simulink model "second_graph_oct9"  (R2026a)
settings: Solver=VariableStepAuto
libraries: fl_lib x10, nesl_utility x7
settings Model: Creator=cathynguyen  LastModifiedBy=cathynguyen

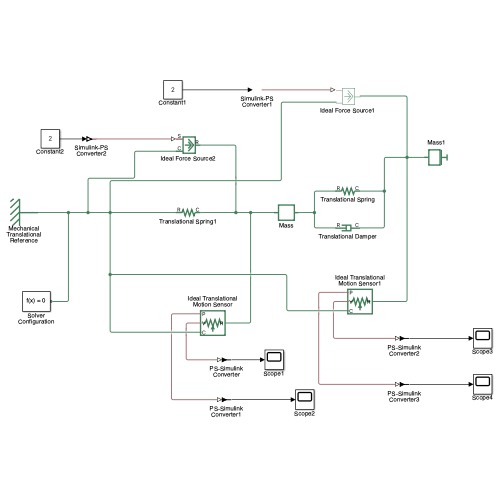
[thumbnail: Simulink's stored preview of the top-level diagram]
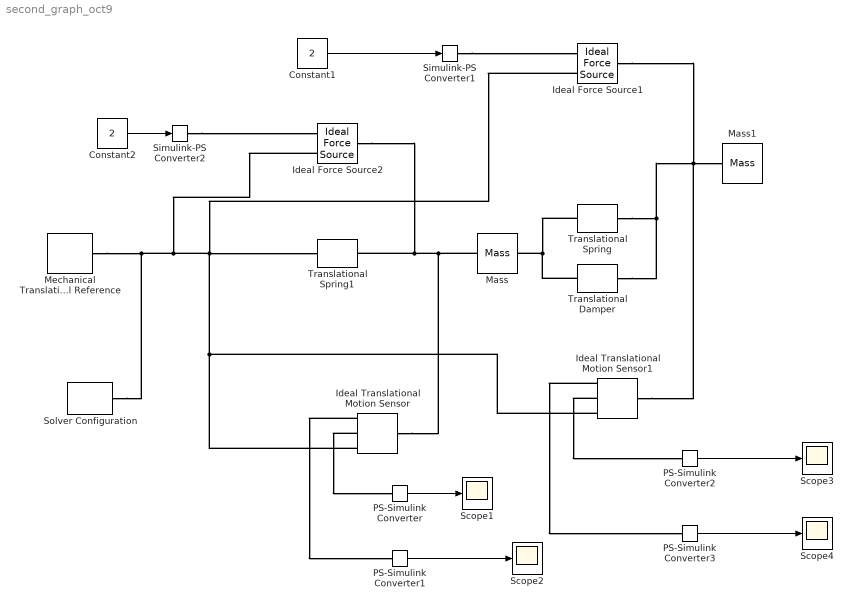
== system second_graph_oct9 ==
  Constant1 : Constant  Value=2
  Constant2 : Constant  Value=2
  Ideal Force Source1 : fl_lib/Mechanical/Mechanical Sources/Ideal Force Source
  Ideal Force Source2 : fl_lib/Mechanical/Mechanical Sources/Ideal Force Source
  Ideal Translational Motion Sensor : fl_lib/Mechanical/Mechanical Sensors/Ideal Translational Motion Sensor  reference=foundation.enum.MeasurementReference.difference  acceleration_port=false  velocity_port=true  position_port=true  offset=0 m
  Ideal Translational Motion Sensor1 : fl_lib/Mechanical/Mechanical Sensors/Ideal Translational Motion Sensor  reference=foundation.enum.MeasurementReference.difference  acceleration_port=false  velocity_port=true  position_port=true  offset=0 m
  Mass : fl_lib/Mechanical/Translational Elements/Mass  mass=1 kg  num_ports=foundation.enum.numPorts2.two  v_specify=off  v_priority=High  v=0 m/s  v_nominal_specify=off  v_nominal_value=1  v_nominal_unit=m/s  f_specify=off  f_priority=None  f=0 N  f_nominal_specify=off  f_nominal_value=1  f_nominal_unit=N
  Mass1 : fl_lib/Mechanical/Translational Elements/Mass  mass=1 kg  num_ports=foundation.enum.numPorts2.one  v_specify=off  v_priority=High  v=0 m/s  v_nominal_specify=off  v_nominal_value=1  v_nominal_unit=m/s  f_specify=off  f_priority=None  f=0 N  f_nominal_specify=off  f_nominal_value=1  f_nominal_unit=N
  Mechanical Translational Reference : fl_lib/Mechanical/Translational Elements/Mechanical Translational Reference
  PS-Simulink Converter{,1..3} (4 alike) : nesl_utility/PS-Simulink Converter  PhysicalDomain=network_engine_domain  SubClassName=ps_output  LeftPortType=input  RightPortType=output  PseudoPeriodic=off  Frequencies=[]  VectorFormat=inherit  Unit=inherit  AffineConversion=off
  Scope{1..4} (4 alike) : Scope
      Scope1 settings: ActiveDisplayYMinimum=-0.30842099880867668  ActiveDisplayYMaximum=0.33479419759874257
      Scope2 settings: ActiveDisplayYMinimum=-0.0096024973516981964  ActiveDisplayYMaximum=0.086422476165283785  DataLoggingVariableName=ScopeData2
      Scope3 settings: ActiveDisplayYMinimum=-0.17620504514124602  ActiveDisplayYMaximum=0.20936892673449753  DataLoggingVariableName=ScopeData3
      Scope4 settings: ActiveDisplayYMinimum=-0.011345220082885486  ActiveDisplayYMaximum=0.1021069807459694  DataLoggingVariableName=ScopeData4
  Simulink-PS Converter1 : nesl_utility/Simulink-PS Converter  PhysicalDomain=network_engine_domain  SubClassName=ps_input  LeftPortType=input  RightPortType=output  PseudoPeriodic=off  Frequencies=[]  NoiseDistribution=none  NoiseParameters=[]  Unit=1  AffineConversion=off  FilteringAndDerivatives=provide  SimscapeFilterOrder=1  InputFilterTimeConstant=0.001  UdotUserProvided=0
  Simulink-PS Converter2 : nesl_utility/Simulink-PS Converter  PhysicalDomain=network_engine_domain  SubClassName=ps_input  LeftPortType=input  RightPortType=output  PseudoPeriodic=off  Frequencies=[]  NoiseDistribution=none  NoiseParameters=[]  Unit=1  AffineConversion=off  FilteringAndDerivatives=provide  SimscapeFilterOrder=1  InputFilterTimeConstant=0.001  UdotUserProvided=0
  Solver Configuration : nesl_utility/Solver Configuration  PhysicalDomain=network_engine_domain  SubClassName=solver  LeftPortType=input  RightPortType=generic  Tones=[]  Harmonics=[]  SimulateNoise=off  Profile=off  UseLocalSampling=off  EnableSwitchedLinearOptims=on  FrequencyDomain=off  UseCCode=off  RelTol=0.001  AbsTol=0.001  MinStep=1e-09  ToWorkspace=off  RevertToSquareIcSolve=off  NumHomotopyIterations=100  PhasorMode=off  PhasorModeNumHarmonics=1  ConsistencySolver=NEWTON_XTOL_AFTER_FTOL  CanonicalOrdering=CANONICAL  OptimizeIntermediates=OPTIMIZED  IndexReductionMethod=DerivativeReplacement  DoDC=off  ResidualTolerance=1e-09  ConsistencyTolSource=GLOBAL  ConsistencyAbsTol=0.001  ConsistencyRelTol=0.001  ConsistencyTolFactor=0.001  UseLocalSolver=off  LocalSolverChoice=NE_BACKWARD_EULER_ADVANCER  ResolveIndetEquations=on  FunctionEvalNumThread=1  LocalSolverSampleTime=0.001  DoFixedCost=off  MaxNonlinIter=3  MaxModeIter=2  ComputeImpulses=off  ImpulseIterations=2  LinearAlgebra=auto  LinearAlgebraNumThread=0  EquationFormulation=NE_TIME_EF  DelaysMemoryBudget=1024  AutomaticFiltering=on  FilteringTimeConstant=0.001  PartitionStorageMethod=AS_NEEDED  PartitionMemoryBudget=1024  PartitionMethod=ROBUST  MultibodyUseLocalSolver=off  MultibodyLocalSolverChoice=ODE1  MultibodyLocalSolverSampleTime=0.001
  Translational Damper : fl_lib/Mechanical/Translational Elements/Translational Damper  D=50 N*s/m  v_specify=off  v_priority=None  v=0 m/s  v_nominal_specify=off  v_nominal_value=1  v_nominal_unit=m/s  f_specify=off  f_priority=None  f=0 N  f_nominal_specify=off  f_nominal_value=1  f_nominal_unit=N
  Translational Spring : fl_lib/Mechanical/Translational Elements/Translational Spring  spr_rate=100 N/m  v_specify=off  v_priority=None  v=0 m/s  v_nominal_specify=off  v_nominal_value=1  v_nominal_unit=m/s  f_specify=off  f_priority=None  f=0 N  f_nominal_specify=off  f_nominal_value=1  f_nominal_unit=N  x_specify=off  x_priority=High  x=0 m  x_nominal_specify=off  x_nominal_value=1  x_nominal_unit=m
  Translational Spring1 : fl_lib/Mechanical/Translational Elements/Translational Spring  spr_rate=100 N/m  v_specify=off  v_priority=None  v=0 m/s  v_nominal_specify=off  v_nominal_value=1  v_nominal_unit=m/s  f_specify=off  f_priority=None  f=0 N  f_nominal_specify=off  f_nominal_value=1  f_nominal_unit=N  x_specify=off  x_priority=High  x=0 m  x_nominal_specify=off  x_nominal_value=1  x_nominal_unit=m
  wires:
  Constant1/1 -> Simulink-PS Converter1/1
  Constant2/1 -> Simulink-PS Converter2/1
  PS-Simulink Converter/1 -> Scope1/1
  PS-Simulink Converter1/1 -> Scope2/1
  PS-Simulink Converter2/1 -> Scope3/1
  PS-Simulink Converter3/1 -> Scope4/1
  connections:
  Translational Spring/LConn1 -- Translational Damper/LConn1 -- Mass/LConn1
  Mass/RConn1 -- Ideal Force Source2/LConn1 -- Translational Spring1/RConn1 -- Ideal Translational Motion Sensor/LConn1
  Translational Spring/RConn1 -- Ideal Translational Motion Sensor1/LConn1 -- Ideal Force Source1/LConn1 -- Mass1/LConn1 -- Translational Damper/RConn1
  Mechanical Translational Reference/LConn1 -- Solver Configuration/RConn1 -- Ideal Translational Motion Sensor1/RConn1 -- Ideal Translational Motion Sensor/RConn1 -- Translational Spring1/LConn1 -- Ideal Force Source1/RConn2 -- Ideal Force Source2/RConn2
  Simulink-PS Converter1/RConn1 -- Ideal Force Source1/RConn1
  Simulink-PS Converter2/RConn1 -- Ideal Force Source2/RConn1
  Ideal Translational Motion Sensor/RConn2 -- PS-Simulink Converter/LConn1
  Ideal Translational Motion Sensor/RConn3 -- PS-Simulink Converter1/LConn1
  Ideal Translational Motion Sensor1/RConn2 -- PS-Simulink Converter2/LConn1
  Ideal Translational Motion Sensor1/RConn3 -- PS-Simulink Converter3/LConn1
